simulink model "dpt"  (R2026a)
settings: Solver=ode23t  StopTime=simlength  FixedStep=tc  MaxStep=glb_time.tc  RelTol=1e-4
values from neighbouring files (symbols this model uses):
  afe_pwm_phase_shift_mod1 = 0    [init_model.m]
  glb_time = timing_setup(fpwm_afe, trgo_afe, fpwm_inv, trgo_inv, fpwm_single_phase_inv, trgo_single_phase_inv, fpwm_dab, trgo_dab,      fpwm_psfbc, trgo_psfbc, fpwm_isop_rail, trgo_isop_rail, fpwm_cllc, trgo_cllc, t_measure, tc_factor, tc_decimation, delay_pwm, dead_time_afe,      dead_time_inv, dead_time_single_phase_inv, dead_time_dab, dead_time_psfbc, dead_time_isop_rail, dead_time_cllc)    [init_model.m]
  time_gain_afe_module_1 = 1.0002    [init_model.m]
  time_gain_inv_module_2 = 1.001    [init_model.m]
libraries: fl_lib x18, nesl_utility x11, diode_rr_lib x2, igbt_dyn_lib x2, ee_lib x1, dclink_for_two_levels x1, single_phase_pwm_modulator x1
settings Model: Creator=dbagn  LastModifiedBy=dbagn
settings SolverCC: NumberNewtonIterations=3.0  ZeroCrossControl=DisableAll  SolverResetMethod=Robust
settings SFSimCC: CustomCodeUndefinedFunction=ThrowError  DefaultCustomCodeDeterministicFunctions=All
settings SFSimCC: SimCustomHeaderCode=|
  | #include "rpi.h"
  | #include "rpi_simulink.h"
  | #include "bemf_obsv_load_est.h"
  | #include "bemf_obsv_load_est_simulink.h"
  | #include "dqpll_grid.h"
  | #include "dsmavgflt.h"
  | #include "bemf_obsv.h"
  | #include "bemf_obsv_simulink.h"
  | #include "mavgflt.h"
  | #include "mavgflt_simulink.h"
  | #include "mavgflts.h"
  | #include "mavgflts_simulink.h"
  | #include "sv_pwm_cm.h"
  | #include "dsmavgflt_simulink.h"
  | #include "linear_double_integrator_observer_simulink.h"
  | #include "sv_pwm_cm_simulink.h"
  | #include "dqvector_pi.h"
  | #include "dqpll_grid_simulink.h"
  | #include "first_harmonic_tracker.h"
  | #include "dqvector_pi_simulink.h"
  | #include "first_harmonic_tracker_simulink.h"
  | #include "dqpll_thyr.h"
  | #include "sv_pwm_simulink.h"
  | #include "sv_pwm.h"
  | #include "dqpll_thyr_simulink.h"
  | #include "linear_double_integrator_observer.h"
  | #include "math_f.h"
settings SFSimCC: SimUserSources=|
  | "rpi.c"
  | "rpi_simulink.c"
  | "mavgflt_simulink.c"
  | "mavgflt.c"
  | "mavgflts_simulink.c"
  | "mavgflts.c"
  | "dsmavgflt_simulink.c"
  | "dsmavgflt.c"
  | "bemf_obsv_simulink.c"
  | "bemf_obsv.c"
  | "bemf_obsv_load_est_simulink.c"
  | "bemf_obsv_load_est.c"
  | "dqvector_pi.c"
  | "dqvector_pi_simulink.c"
  | "sv_pwm_simulink.c"
  | "sv_pwm.c"
  | "first_harmonic_tracker_simulink.c"
  | "first_harmonic_tracker.c"
  | "dqpll_thyr_simulink.c"
  | "dqpll_thyr.c"
  | "dqpll_grid_simulink.c"
  | "dqpll_grid.c"
  | "linear_double_integrator_observer_simulink.c"
  | "linear_double_integrator_observer.c"
  | "sv_pwm_cm_simulink.c"
  | "sv_pwm_cm.c"
settings SFSimCC: SimUserIncludeDirs=|
  | include
  | src
settings SimscapeCC: SimscapeNominalValues="[{\"value\":\"1\",\"unit\":\"A\"},{\"value\":\"1\",\"unit\":\"bar\"},{\"value\":\"1\",\"unit\":\"cm^2\"},{\"value\":\"1\",\"unit\":\"cm^3/s\"},{\"value\":\"1\",\"unit\":\"kJ/kg\"},{\"value\":\"1\",\"unit\":\"kW\"},{\"value\":\"1\",\"unit\":\"l\"},{\"value\":\"1\",\"unit\":\"N\"},{\"value\":\"1\",\"unit\":\"N*m\"},{\"value\":\"1\",\"unit\":\"V\"}]"  SimscapeLogType=none  SimscapeLogDataHistory=5000.0

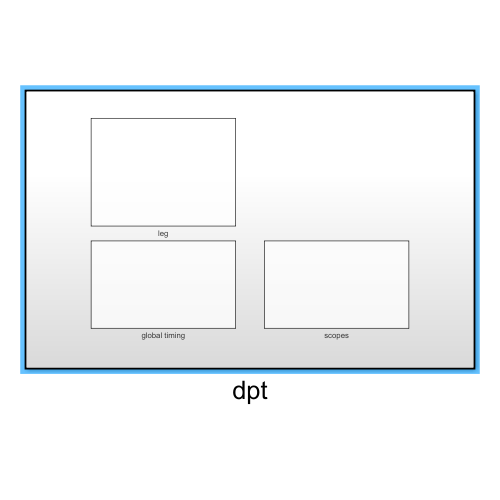
[thumbnail: Simulink's stored preview of the top-level diagram]
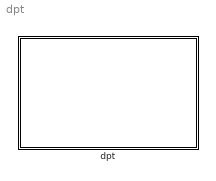
== system dpt ==
  dpt : Subsystem

== system dpt/dpt ==
  global timing : Subsystem
  leg : Subsystem
  scopes : Subsystem

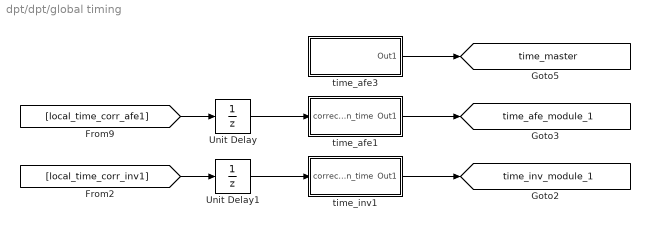
== system dpt/dpt/global timing ==
  Unit Delay : UnitDelay  SampleTime=glb_time.tc
  Unit Delay1 : UnitDelay  SampleTime=glb_time.tc
  time_afe1 : Subsystem  mask{k=time_gain_afe_module_1}
      mask prompts: k "Time Gain"
      mask Display:
      | disp('time-gen');
      | port_label('input', 1, 'crt');
      | port_label('output', 1, 'tout');
  time_afe3 : Subsystem  mask{k=1}
      mask prompts: k "Time Gain"
      mask Display:
      | disp('time-gen');
      | port_label('output', 1, 'tout');
  time_inv1 : Subsystem  mask{k=time_gain_inv_module_2}
      mask prompts: k "Time Gain"
      mask Display:
      | disp('time-gen');
      | port_label('input', 1, 'crt');
      | port_label('output', 1, 'tout');
  tag scope: time_afe_module_1=global, time_inv_module_1=global, time_master=global
  wires:
  Unit Delay1/1 -> time_inv1/1(correction_time)
  [local_time_corr_inv1] -> Unit Delay1/1
  Unit Delay/1 -> time_afe1/1(correction_time)
  [local_time_corr_afe1] -> Unit Delay/1
  time_afe3/1(Out1) -> [time_master]
  time_inv1/1(Out1) -> [time_inv_module_1]
  time_afe1/1(Out1) -> [time_afe_module_1]

== system dpt/dpt/leg ==
  Electrical Reference : fl_lib/Electrical/Electrical Elements/Electrical Reference
  Inductor : fl_lib/Electrical/Electrical Elements/Inductor  l=50e-6 H  r=0 Ohm  g=1e-9 1/Ohm  i_specify=off  i_priority=None  i=0 A  i_nominal_specify=off  i_nominal_value=1  i_nominal_unit=A  v_specify=off  v_priority=None  v=0 V  v_nominal_specify=off  v_nominal_value=1  v_nominal_unit=V  i_L_specify=off  i_L_priority=High  i_L=0 A  i_L_nominal_specify=off  i_L_nominal_value=1  i_L_nominal_unit=A
  Solver Configuration : nesl_utility/Solver Configuration  PhysicalDomain=network_engine_domain  SubClassName=solver  LeftPortType=input  RightPortType=generic  Tones=[]  Harmonics=[]  SimulateNoise=off  Profile=off  UseLocalSampling=off  EnableSwitchedLinearOptims=on  FrequencyDomain=off  UseCCode=off  RelTol=0.001  AbsTol=0.001  MinStep=1e-09  ToWorkspace=off  RevertToSquareIcSolve=off  NumHomotopyIterations=100  PhasorMode=off  PhasorModeNumHarmonics=1  ConsistencySolver=NEWTON_XTOL_AFTER_FTOL  CanonicalOrdering=CANONICAL  OptimizeIntermediates=OPTIMIZED  IndexReductionMethod=DerivativeReplacement  DoDC=off  ResidualTolerance=1e-09  ConsistencyTolSource=GLOBAL  ConsistencyAbsTol=0.001  ConsistencyRelTol=0.001  ConsistencyTolFactor=0.001  UseLocalSolver=off  LocalSolverChoice=NE_BACKWARD_EULER_ADVANCER  ResolveIndetEquations=on  FunctionEvalNumThread=1  LocalSolverSampleTime=glb_time.tc  DoFixedCost=off  MaxNonlinIter=nonlinear_iterations  MaxModeIter=2  ComputeImpulses=off  ImpulseIterations=2  LinearAlgebra=auto  LinearAlgebraNumThread=0  EquationFormulation=NE_TIME_EF  DelaysMemoryBudget=1024  AutomaticFiltering=on  FilteringTimeConstant=0.001  PartitionStorageMethod=AS_NEEDED  PartitionMemoryBudget=1024  PartitionMethod=ROBUST  MultibodyUseLocalSolver=off  MultibodyLocalSolverChoice=ODE1  MultibodyLocalSolverSampleTime=0.001
  Voltage Source : ee_lib/Sources/Voltage Source  dc_voltage=1070 V  ac_voltage=0 V  ac_shift=0 rad  ac_frequency=60 Hz  noise_mode=ee.enum.sources.noise.Disabled  PSD=0 V^2/Hz  sample_time=1e-3 s  repeatability=ee.enum.sources.repeatability.NotRepeatable  user_seed=0  auto_seed=2780181638  i_specify=off  i_priority=None  i=0 A  i_nominal_specify=off  i_nominal_value=1  i_nominal_unit=A  v_specify=off  v_priority=None  v=0 V  v_nominal_specify=off  v_nominal_value=1  v_nominal_unit=V
  leg : Subsystem
  connections:
  Voltage Source/RConn1 -- Solver Configuration/RConn1 -- Electrical Reference/LConn1 -- leg/RConn2
  Voltage Source/LConn1 -- leg/RConn1
  Inductor/LConn1 -- leg/LConn1
  Inductor/RConn1 -- leg/LConn2

== system dpt/dpt/scopes ==
  igbt_dyn : Subsystem

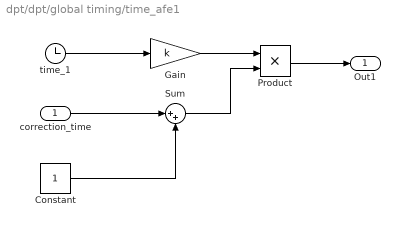
== system dpt/dpt/global timing/time_afe1 ==
  correction_time : Inport
  Constant : Constant
  Gain : Gain  Gain=k
  Product : Product
  Sum : Sum  Inputs=|++
  time_1 : Clock
  Out1 : Outport
  wires:
  Constant/1 -> Sum/2
  Sum/1 -> Product/2
  correction_time/1 -> Sum/1
  Product/1 -> Out1/1
  Gain/1 -> Product/1
  time_1/1 -> Gain/1

== system dpt/dpt/global timing/time_afe3 ==
  Gain : Gain  Gain=k
  time_1 : Clock
  Out1 : Outport
  wires:
  time_1/1 -> Gain/1
  Gain/1 -> Out1/1

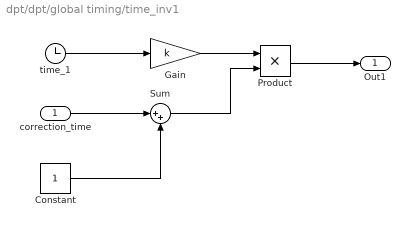
== system dpt/dpt/global timing/time_inv1 ==
  correction_time : Inport
  Constant : Constant
  Gain : Gain  Gain=k
  Product : Product
  Sum : Sum  Inputs=|++
  time_1 : Clock
  Out1 : Outport
  wires:
  Sum/1 -> Product/2
  Constant/1 -> Sum/2
  correction_time/1 -> Sum/1
  Product/1 -> Out1/1
  Gain/1 -> Product/1
  time_1/1 -> Gain/1

== system dpt/dpt/leg/leg ==
  dclink : Subsystem
  leg_pwm : Subsystem
  leg_with_igbt_dyn : Subsystem
  u1 : PMIOPort  Side=Left
  u2 : PMIOPort  Port=2  Side=Left
  Udc(+) : PMIOPort  Port=3  Side=Right
  Udc(-) : PMIOPort  Port=4  Side=Right
  wires:
  leg_pwm/1(gate_cmds) -> leg_with_igbt_dyn/1(gate_commands)
  connections:
  leg_with_igbt_dyn/RConn1 -- u1/RConn1
  leg_with_igbt_dyn/RConn2 -- u2/RConn1
  dclink/RConn1 -- Udc(+)/RConn1
  dclink/LConn1 -- leg_with_igbt_dyn/LConn1
  dclink/LConn2 -- leg_with_igbt_dyn/LConn2
  dclink/RConn2 -- Udc(-)/RConn1

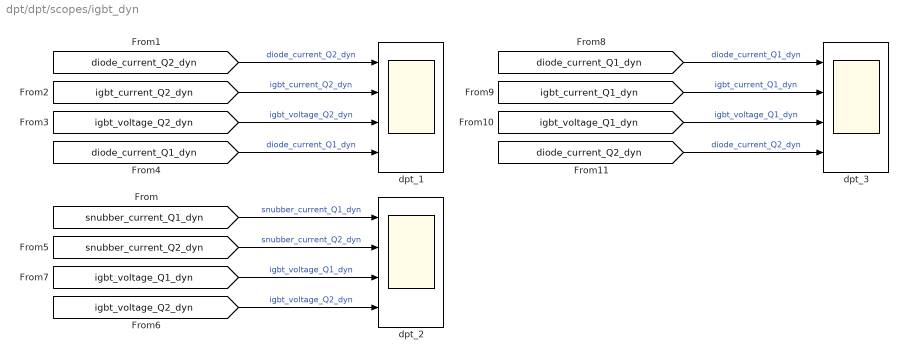
== system dpt/dpt/scopes/igbt_dyn ==
  dpt_1 : Scope  NumInputPorts=4
      settings: SampleTime=glb_time.tc  ActiveDisplayString=3  ActiveDisplayYMinimum=-199.00170924097591  ActiveDisplayYMaximum=1779.7216480499278
  dpt_2 : Scope  NumInputPorts=4
      settings: SampleTime=glb_time.tc  ActiveDisplayString=3  ActiveDisplayYMinimum=-153.38142747263524  ActiveDisplayYMaximum=1358.8196055613325
  dpt_3 : Scope  NumInputPorts=4
      settings: SampleTime=glb_time.tc  ActiveDisplayString=3  ActiveDisplayYMinimum=-153.38142747263524  ActiveDisplayYMaximum=1358.8196055613325  DataLoggingVariableName=ScopeData2
  wires:
  [diode_current_Q2_dyn] -> dpt_1/1  "diode_current_Q2_dyn"
  [igbt_voltage_Q2_dyn] -> dpt_1/3  "igbt_voltage_Q2_dyn"
  [igbt_current_Q2_dyn] -> dpt_1/2  "igbt_current_Q2_dyn"
  [diode_current_Q1_dyn] -> dpt_1/4  "diode_current_Q1_dyn"
  [snubber_current_Q1_dyn] -> dpt_2/1  "snubber_current_Q1_dyn"
  [snubber_current_Q2_dyn] -> dpt_2/2  "snubber_current_Q2_dyn"
  [igbt_voltage_Q2_dyn] -> dpt_2/4  "igbt_voltage_Q2_dyn"
  [igbt_voltage_Q1_dyn] -> dpt_2/3  "igbt_voltage_Q1_dyn"
  [diode_current_Q2_dyn] -> dpt_3/4  "diode_current_Q2_dyn"
  [igbt_current_Q1_dyn] -> dpt_3/2  "igbt_current_Q1_dyn"
  [igbt_voltage_Q1_dyn] -> dpt_3/3  "igbt_voltage_Q1_dyn"
  [diode_current_Q1_dyn] -> dpt_3/1  "diode_current_Q1_dyn"

== system dpt/dpt/leg/leg/dclink ==
  dclink1 : dclink_for_two_levels/dclink  Cdc=hwdata.afe.CFi  Rudc_measure=1e6  Vdc_scale=hwdata.afe.udc_nom
  Udc(+) : PMIOPort  Side=Right
  udc(+) : PMIOPort  Port=2  Side=Left
  udc(-) : PMIOPort  Port=3  Side=Left
  Udc(-) : PMIOPort  Port=4  Side=Right
  connections:
  dclink1/LConn2 -- udc(-)/RConn1
  dclink1/RConn2 -- Udc(-)/RConn1
  dclink1/RConn1 -- Udc(+)/RConn1
  dclink1/LConn1 -- udc(+)/RConn1

== system dpt/dpt/leg/leg/leg_pwm ==
  Constant1 : Constant  Value=afe_pwm_phase_shift_mod1
  Constant2 : Constant  Value=0.5
  modulator1 : Subsystem
  td2tc_1 : TransferFcn  Denominator=[glb_time.tc 1]
  gate_cmds : Outport
  wires:
  td2tc_1/1 -> modulator1/1(u)  "du(t)"
  Constant2/1 -> td2tc_1/1
  Constant1/1 -> modulator1/2(phase)
  modulator1/1(gate_cmds) -> gate_cmds/1

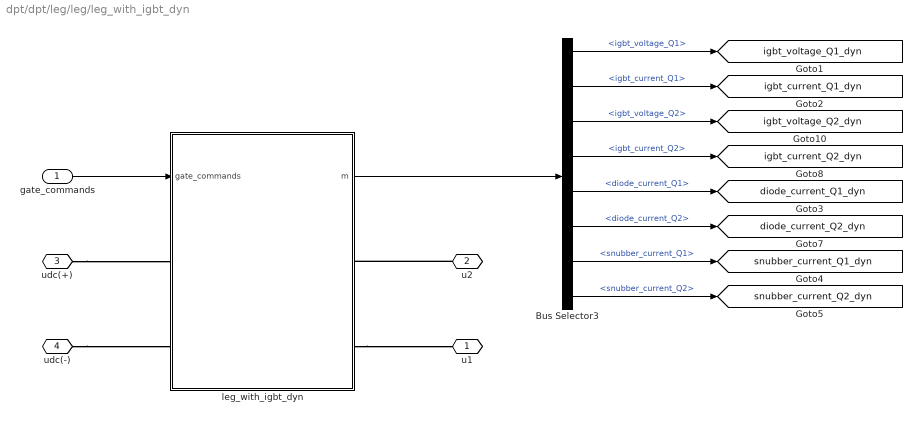
== system dpt/dpt/leg/leg/leg_with_igbt_dyn ==
  gate_commands : Inport
  Bus Selector3 : BusSelector  OutputSignals=igbt_voltage_Q1,igbt_current_Q1,igbt_voltage_Q2,igbt_current_Q2,diode_current_Q1,diode_current_Q2,snubber_current_Q1,snubber_current_Q2
  leg_with_igbt_dyn : Subsystem
  u1 : PMIOPort  Side=Right
  u2 : PMIOPort  Port=2  Side=Right
  udc(+) : PMIOPort  Port=3  Side=Left
  udc(-) : PMIOPort  Port=4  Side=Left
  tag scope: diode_current_Q1_dyn=global, diode_current_Q2_dyn=global, igbt_current_Q1_dyn=global, igbt_current_Q2_dyn=global, igbt_voltage_Q1_dyn=global, igbt_voltage_Q2_dyn=global, snubber_current_Q1_dyn=global, snubber_current_Q2_dyn=global
  wires:
  Bus Selector3/6 -> [diode_current_Q2_dyn]  "<diode_current_Q2>"
  Bus Selector3/5 -> [diode_current_Q1_dyn]  "<diode_current_Q1>"
  Bus Selector3/4 -> [igbt_current_Q2_dyn]  "<igbt_current_Q2>"
  Bus Selector3/3 -> [igbt_voltage_Q2_dyn]  "<igbt_voltage_Q2>"
  Bus Selector3/2 -> [igbt_current_Q1_dyn]  "<igbt_current_Q1>"
  Bus Selector3/1 -> [igbt_voltage_Q1_dyn]  "<igbt_voltage_Q1>"
  gate_commands/1 -> leg_with_igbt_dyn/1(gate_commands)
  leg_with_igbt_dyn/1(m) -> Bus Selector3/1
  Bus Selector3/7 -> [snubber_current_Q1_dyn]  "<snubber_current_Q1>"
  Bus Selector3/8 -> [snubber_current_Q2_dyn]  "<snubber_current_Q2>"
  connections:
  u2/RConn1 -- leg_with_igbt_dyn/RConn1
  udc(-)/RConn1 -- leg_with_igbt_dyn/LConn2
  udc(+)/RConn1 -- leg_with_igbt_dyn/LConn1
  leg_with_igbt_dyn/RConn2 -- u1/RConn1

== system dpt/dpt/leg/leg/leg_pwm/modulator1 ==
  u : Inport
  phase : Inport  Port=2
  one phase PWM generator with global TRGO : Subsystem  mask{f=glb_time.fPWM_AFE, m_up=0.98, m_low=0.02, dead_time=glb_time.dead_time_AFE, pos_cmd_gate=15, neg_cmd_gate=-8, polarity=1, tc=glb_time.tc, double_sampling=glb_time.TRGO_AFE_double_update}
      mask prompts: f "Frequency (Hz)"; m_up "Max Input Modulation Value"; m_low "Min Input Modulation Value"; dead_time "Dead Time (s)"; pos_cmd_gate "Positive Gate Voltage (V)"; neg_cmd_gate "Negative Gate Voltage (V)"; polarity "Polarity (pu)"; tc "Sampling time"
  gate_cmds : Outport
  wires:
  one phase PWM generator with global TRGO/2(gate_cmds) -> gate_cmds/1
  phase/1 -> one phase PWM generator with global TRGO/2(phase)
  u/1 -> one phase PWM generator with global TRGO/3(m)
  [time_afe_module_1] -> one phase PWM generator with global TRGO/1(time_source)

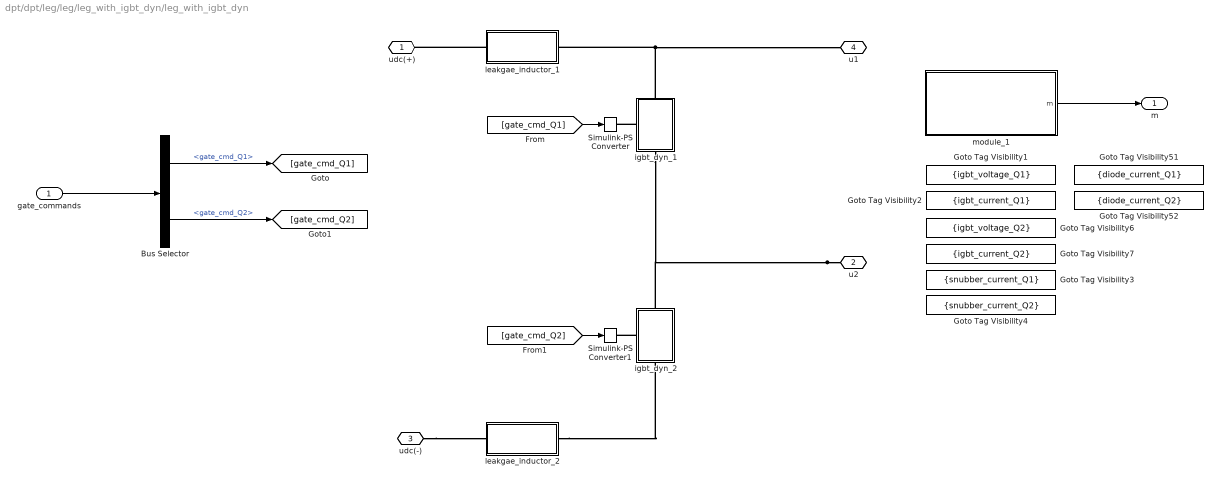
== system dpt/dpt/leg/leg/leg_with_igbt_dyn/leg_with_igbt_dyn ==
  gate_commands : Inport
  Bus Selector : BusSelector  OutputSignals=gate_cmd_Q1,gate_cmd_Q2
  Goto Tag Visibility1 : GotoTagVisibility  GotoTag=igbt_voltage_Q1
  Goto Tag Visibility2 : GotoTagVisibility  GotoTag=igbt_current_Q1
  Goto Tag Visibility3 : GotoTagVisibility  GotoTag=snubber_current_Q1
  Goto Tag Visibility4 : GotoTagVisibility  GotoTag=snubber_current_Q2
  Goto Tag Visibility51 : GotoTagVisibility  GotoTag=diode_current_Q1
  Goto Tag Visibility52 : GotoTagVisibility  GotoTag=diode_current_Q2
  Goto Tag Visibility6 : GotoTagVisibility  GotoTag=igbt_voltage_Q2
  Goto Tag Visibility7 : GotoTagVisibility  GotoTag=igbt_current_Q2
  Simulink-PS Converter : nesl_utility/Simulink-PS Converter  PhysicalDomain=network_engine_domain  SubClassName=ps_input  LeftPortType=input  RightPortType=output  PseudoPeriodic=off  Frequencies=[]  NoiseDistribution=none  NoiseParameters=[]  Unit=V  AffineConversion=off  FilteringAndDerivatives=provide  SimscapeFilterOrder=1  InputFilterTimeConstant=0.001  UdotUserProvided=0
  Simulink-PS Converter1 : nesl_utility/Simulink-PS Converter  PhysicalDomain=network_engine_domain  SubClassName=ps_input  LeftPortType=input  RightPortType=output  PseudoPeriodic=off  Frequencies=[]  NoiseDistribution=none  NoiseParameters=[]  Unit=V  AffineConversion=off  FilteringAndDerivatives=provide  SimscapeFilterOrder=1  InputFilterTimeConstant=0.001  UdotUserProvided=0
  igbt_dyn_1 : Subsystem
      settings: PortSchema="{\"entries\":[{\"content\":{\"sides\":[{\"content\":{\"connectorIds\":[\"LConn1\"]},\"type\":\"ConnectorPlacement.EquallySpacedRectSide\",\"uuid\":\"9277da8d-d460-43e6-8478-dd662f15d226\"},{\"content\":{\"connectorIds\":[],\"side\":\"RIGHT\"},\"type\":\"ConnectorPlacement.EquallySpacedRectSide\",\"uuid\":\"a7ece396-f1d9-4f4f-a05b-db1fc65d6e1d\"},{\"content\":{\"connectorIds\":[\"LConn2\"],\"side\":\"TOP\"},\"type\":\"ConnectorPlacement.EquallySpacedRectSide\",\"uuid\":\"fdd70777-e9cf-4317-afb6-cae87f75d5b0\"},{\"content\":{\"connectorIds\":[\"RConn1\"],\"side\":\"BOTTOM\"},\"type\":\"ConnectorPlacement.EquallySpacedRectSide\",\"uuid\":\"2353ed68-b1a1-4775-9ca9-31e268d5443b\"}]},\"type\":\"ConnectorPlacement.EquallySpacedConnector\",\"uuid\":\"d5479f4c-4e65-4791-adcb-73df11f88590\"}],\"packageUris\":[\"http://schema.mathworks.com/mf0/Connector/R2020b\"],\"version\":\"1.0\"}"
  igbt_dyn_2 : Subsystem
      settings: PortSchema="{\"entries\":[{\"content\":{\"sides\":[{\"content\":{\"connectorIds\":[\"LConn1\"]},\"type\":\"ConnectorPlacement.EquallySpacedRectSide\",\"uuid\":\"9277da8d-d460-43e6-8478-dd662f15d226\"},{\"content\":{\"connectorIds\":[],\"side\":\"RIGHT\"},\"type\":\"ConnectorPlacement.EquallySpacedRectSide\",\"uuid\":\"a7ece396-f1d9-4f4f-a05b-db1fc65d6e1d\"},{\"content\":{\"connectorIds\":[\"LConn2\"],\"side\":\"TOP\"},\"type\":\"ConnectorPlacement.EquallySpacedRectSide\",\"uuid\":\"fdd70777-e9cf-4317-afb6-cae87f75d5b0\"},{\"content\":{\"connectorIds\":[\"RConn1\"],\"side\":\"BOTTOM\"},\"type\":\"ConnectorPlacement.EquallySpacedRectSide\",\"uuid\":\"2353ed68-b1a1-4775-9ca9-31e268d5443b\"}]},\"type\":\"ConnectorPlacement.EquallySpacedConnector\",\"uuid\":\"d5479f4c-4e65-4791-adcb-73df11f88590\"}],\"packageUris\":[\"http://schema.mathworks.com/mf0/Connector/R2020b\"],\"version\":\"1.0\"}"
  leakgae_inductor_1 : Subsystem
  leakgae_inductor_2 : Subsystem
  module_1 : Subsystem
  udc(+) : PMIOPort  Side=Left
  u2 : PMIOPort  Port=2  Side=Right
  udc(-) : PMIOPort  Port=3  Side=Left
  u1 : PMIOPort  Port=4  Side=Right
  m : Outport
  wires:
  module_1/1(m) -> m/1
  Bus Selector/2 -> [gate_cmd_Q2]  "<gate_cmd_Q2>"
  Bus Selector/1 -> [gate_cmd_Q1]  "<gate_cmd_Q1>"
  [gate_cmd_Q2] -> Simulink-PS Converter1/1
  [gate_cmd_Q1] -> Simulink-PS Converter/1
  gate_commands/1 -> Bus Selector/1
  connections:
  igbt_dyn_2/LConn1 -- Simulink-PS Converter1/RConn1
  igbt_dyn_1/LConn1 -- Simulink-PS Converter/RConn1
  u2/RConn1 -- igbt_dyn_1/RConn1 -- igbt_dyn_2/LConn2
  leakgae_inductor_2/RConn1 -- igbt_dyn_2/RConn1
  igbt_dyn_1/LConn2 -- leakgae_inductor_1/RConn1 -- u1/RConn1
  udc(-)/RConn1 -- leakgae_inductor_2/LConn1
  leakgae_inductor_1/LConn1 -- udc(+)/RConn1

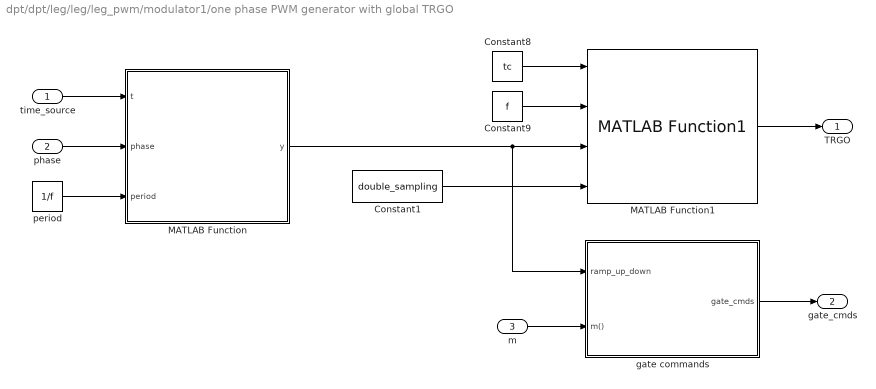
== system dpt/dpt/leg/leg/leg_pwm/modulator1/one phase PWM generator with global TRGO ==
  time_source : Inport
  phase : Inport  Port=2
  m : Inport  Port=3
  Constant1 : Constant  Value=double_sampling
  Constant8 : Constant  Value=tc
  Constant9 : Constant  Value=f
  MATLAB Function : MATLAB Function  TreatAsAtomicUnit=on  SystemSampleTime=tc
  MATLAB Function1 : single_phase_pwm_modulator/Single phase two level PWM generator with global TRGO/MATLAB Function1  SystemSampleTime=tc  VariantActivationTime=update diagram  EmptyChoice=off  PassThrough=off  PassThroughVariantControl=(default)  EmptyChoiceVariantControl=(default)  AllowFlexibleInterface=on  Latency=0  AutoFrameSizeCalculation=off
  gate commands : Subsystem
  period : Constant  Value=1/f
  TRGO : Outport
  gate_cmds : Outport  Port=2
  wires:
  period/1 -> MATLAB Function/3(period)
  phase/1 -> MATLAB Function/2(phase)
  MATLAB Function/1(y) -> gate commands/1(ramp_up_down), MATLAB Function1/3
  MATLAB Function1/1 -> TRGO/1
  Constant8/1 -> MATLAB Function1/1
  Constant9/1 -> MATLAB Function1/2
  m/1 -> gate commands/2(m())
  gate commands/1(gate_cmds) -> gate_cmds/1
  time_source/1 -> MATLAB Function/1(t)
  Constant1/1 -> MATLAB Function1/4

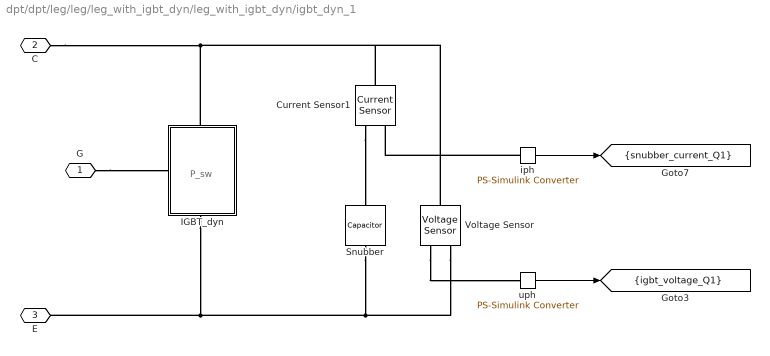
== system dpt/dpt/leg/leg/leg_with_igbt_dyn/leg_with_igbt_dyn/igbt_dyn_1 ==
  note: P_sw
  Current Sensor1 : fl_lib/Electrical/Electrical Sensors/Current Sensor
  IGBT_dyn : Subsystem
      settings: PortSchema="{\"entries\":[{\"content\":{\"sides\":[{\"content\":{\"connectorIds\":[\"LConn1\"]},\"type\":\"ConnectorPlacement.EquallySpacedRectSide\",\"uuid\":\"c3d88d60-081d-4221-ab18-079856838dba\"},{\"content\":{\"side\":\"RIGHT\"},\"type\":\"ConnectorPlacement.EquallySpacedRectSide\",\"uuid\":\"76e7d76c-8b60-4107-8aac-a7654bd886e1\"},{\"content\":{\"connectorIds\":[\"LConn2\"],\"side\":\"TOP\"},\"type\":\"ConnectorPlacement.EquallySpacedRectSide\",\"uuid\":\"fbef57e1-7143-4076-ada8-0654b1d9ee0b\"},{\"content\":{\"connectorIds\":[\"RConn1\"],\"side\":\"BOTTOM\"},\"type\":\"ConnectorPlacement.EquallySpacedRectSide\",\"uuid\":\"f2fea5db-9515-452a-a480-7d54bae36c49\"}]},\"type\":\"ConnectorPlacement.EquallySpacedConnector\",\"uuid\":\"cddff0b8-236e-4840-ad87-03abcdd65fe7\"}],\"packageUris\":[\"http://schema.mathworks.com/mf0/Connector/R2020b\"],\"version\":\"1.0\"}"
  Snubber : fl_lib/Electrical/Electrical Elements/Capacitor  c=igbt.afe.Csnubber_zvs F  r=igbt.afe.Rsnubber_zvs Ohm  g=0 1/Ohm  i_specify=off  i_priority=None  i=0 A  i_nominal_specify=off  i_nominal_value=1  i_nominal_unit=A  v_specify=off  v_priority=None  v=0 V  v_nominal_specify=off  v_nominal_value=1  v_nominal_unit=V  vc_specify=off  vc_priority=High  vc=0 V  vc_nominal_specify=off  vc_nominal_value=1  vc_nominal_unit=V
  Voltage Sensor : fl_lib/Electrical/Electrical Sensors/Voltage Sensor
  iph : nesl_utility/PS-Simulink Converter  PhysicalDomain=network_engine_domain  SubClassName=ps_output  LeftPortType=input  RightPortType=output  PseudoPeriodic=off  Frequencies=[]  VectorFormat=1-D array  Unit=A  AffineConversion=off
  uph : nesl_utility/PS-Simulink Converter  PhysicalDomain=network_engine_domain  SubClassName=ps_output  LeftPortType=input  RightPortType=output  PseudoPeriodic=off  Frequencies=[]  VectorFormat=1-D array  Unit=V  AffineConversion=off
  G : PMIOPort  Side=Left
  C : PMIOPort  Port=2  Side=Left
  E : PMIOPort  Port=3  Side=Right
  tag scope: igbt_voltage_Q1=scoped, snubber_current_Q1=scoped
  wires:
  uph/1 -> [igbt_voltage_Q1]
  iph/1 -> [snubber_current_Q1]
  connections:
  G/RConn1 -- IGBT_dyn/LConn1
  Voltage Sensor/RConn1 -- uph/LConn1
  IGBT_dyn/LConn2 -- Current Sensor1/LConn1 -- Voltage Sensor/LConn1 -- C/RConn1
  Voltage Sensor/RConn2 -- Snubber/RConn1 -- E/RConn1 -- IGBT_dyn/RConn1
  Current Sensor1/RConn2 -- Snubber/LConn1
  iph/LConn1 -- Current Sensor1/RConn1

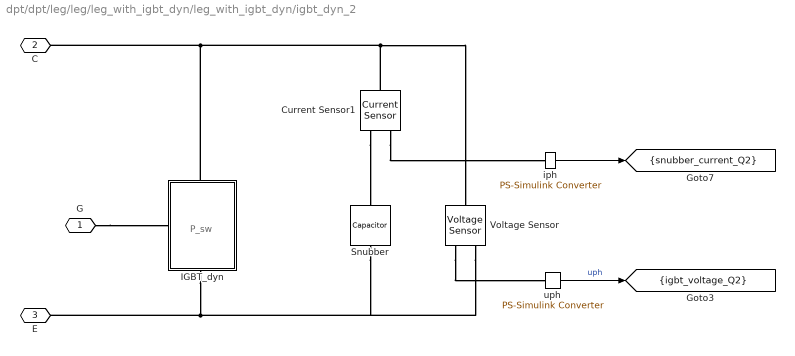
== system dpt/dpt/leg/leg/leg_with_igbt_dyn/leg_with_igbt_dyn/igbt_dyn_2 ==
  note: P_sw
  Current Sensor1 : fl_lib/Electrical/Electrical Sensors/Current Sensor
  IGBT_dyn : Subsystem
      settings: PortSchema="{\"entries\":[{\"content\":{\"sides\":[{\"content\":{\"connectorIds\":[\"LConn1\"]},\"type\":\"ConnectorPlacement.EquallySpacedRectSide\",\"uuid\":\"c3d88d60-081d-4221-ab18-079856838dba\"},{\"content\":{\"side\":\"RIGHT\"},\"type\":\"ConnectorPlacement.EquallySpacedRectSide\",\"uuid\":\"76e7d76c-8b60-4107-8aac-a7654bd886e1\"},{\"content\":{\"connectorIds\":[\"LConn2\"],\"side\":\"TOP\"},\"type\":\"ConnectorPlacement.EquallySpacedRectSide\",\"uuid\":\"fbef57e1-7143-4076-ada8-0654b1d9ee0b\"},{\"content\":{\"connectorIds\":[\"RConn1\"],\"side\":\"BOTTOM\"},\"type\":\"ConnectorPlacement.EquallySpacedRectSide\",\"uuid\":\"f2fea5db-9515-452a-a480-7d54bae36c49\"}]},\"type\":\"ConnectorPlacement.EquallySpacedConnector\",\"uuid\":\"cddff0b8-236e-4840-ad87-03abcdd65fe7\"}],\"packageUris\":[\"http://schema.mathworks.com/mf0/Connector/R2020b\"],\"version\":\"1.0\"}"
  Snubber : fl_lib/Electrical/Electrical Elements/Capacitor  c=igbt.afe.Csnubber_zvs F  r=igbt.afe.Rsnubber_zvs Ohm  g=0 1/Ohm  i_specify=off  i_priority=None  i=0 A  i_nominal_specify=off  i_nominal_value=1  i_nominal_unit=A  v_specify=off  v_priority=None  v=0 V  v_nominal_specify=off  v_nominal_value=1  v_nominal_unit=V  vc_specify=off  vc_priority=High  vc=0 V  vc_nominal_specify=off  vc_nominal_value=1  vc_nominal_unit=V
  Voltage Sensor : fl_lib/Electrical/Electrical Sensors/Voltage Sensor
  iph : nesl_utility/PS-Simulink Converter  PhysicalDomain=network_engine_domain  SubClassName=ps_output  LeftPortType=input  RightPortType=output  PseudoPeriodic=off  Frequencies=[]  VectorFormat=1-D array  Unit=A  AffineConversion=off
  uph : nesl_utility/PS-Simulink Converter  PhysicalDomain=network_engine_domain  SubClassName=ps_output  LeftPortType=input  RightPortType=output  PseudoPeriodic=off  Frequencies=[]  VectorFormat=1-D array  Unit=V  AffineConversion=off
  G : PMIOPort  Side=Left
  C : PMIOPort  Port=2  Side=Left
  E : PMIOPort  Port=3  Side=Right
  tag scope: igbt_voltage_Q2=scoped, snubber_current_Q2=scoped
  wires:
  uph/1 -> [igbt_voltage_Q2]  "uph"
  iph/1 -> [snubber_current_Q2]
  connections:
  IGBT_dyn/RConn1 -- Voltage Sensor/RConn2 -- Snubber/RConn1 -- E/RConn1
  Voltage Sensor/RConn1 -- uph/LConn1
  G/RConn1 -- IGBT_dyn/LConn1
  Current Sensor1/RConn2 -- Snubber/LConn1
  Current Sensor1/RConn1 -- iph/LConn1
  Current Sensor1/LConn1 -- Voltage Sensor/LConn1 -- IGBT_dyn/LConn2 -- C/RConn1

== system dpt/dpt/leg/leg/leg_with_igbt_dyn/leg_with_igbt_dyn/leakgae_inductor_1 ==
  Inductor : fl_lib/Electrical/Electrical Elements/Inductor  l=10e-9 H  r=5e-3 Ohm  g=1e-9 1/Ohm  i_specify=off  i_priority=None  i=0 A  i_nominal_specify=off  i_nominal_value=1  i_nominal_unit=A  v_specify=off  v_priority=None  v=0 V  v_nominal_specify=off  v_nominal_value=1  v_nominal_unit=V  i_L_specify=off  i_L_priority=High  i_L=0 A  i_L_nominal_specify=off  i_L_nominal_value=1  i_L_nominal_unit=A
  Resistor : fl_lib/Electrical/Electrical Elements/Resistor  R=1 Ohm  i_specify=off  i_priority=None  i=0 A  i_nominal_specify=off  i_nominal_value=1  i_nominal_unit=A  v_specify=off  v_priority=None  v=0 V  v_nominal_specify=off  v_nominal_value=1  v_nominal_unit=V
  in : PMIOPort  Side=Left
  out : PMIOPort  Port=2  Side=Right
  connections:
  Resistor/RConn1 -- Inductor/RConn1 -- out/RConn1
  Resistor/LConn1 -- Inductor/LConn1 -- in/RConn1

== system dpt/dpt/leg/leg/leg_with_igbt_dyn/leg_with_igbt_dyn/leakgae_inductor_2 ==
  Inductor : fl_lib/Electrical/Electrical Elements/Inductor  l=10e-9 H  r=5e-3 Ohm  g=1e-9 1/Ohm  i_specify=off  i_priority=None  i=0 A  i_nominal_specify=off  i_nominal_value=1  i_nominal_unit=A  v_specify=off  v_priority=None  v=0 V  v_nominal_specify=off  v_nominal_value=1  v_nominal_unit=V  i_L_specify=off  i_L_priority=High  i_L=0 A  i_L_nominal_specify=off  i_L_nominal_value=1  i_L_nominal_unit=A
  Resistor : fl_lib/Electrical/Electrical Elements/Resistor  R=1 Ohm  i_specify=off  i_priority=None  i=0 A  i_nominal_specify=off  i_nominal_value=1  i_nominal_unit=A  v_specify=off  v_priority=None  v=0 V  v_nominal_specify=off  v_nominal_value=1  v_nominal_unit=V
  in : PMIOPort  Side=Left
  out : PMIOPort  Port=2  Side=Right
  connections:
  in/RConn1 -- Inductor/LConn1 -- Resistor/LConn1
  out/RConn1 -- Inductor/RConn1 -- Resistor/RConn1

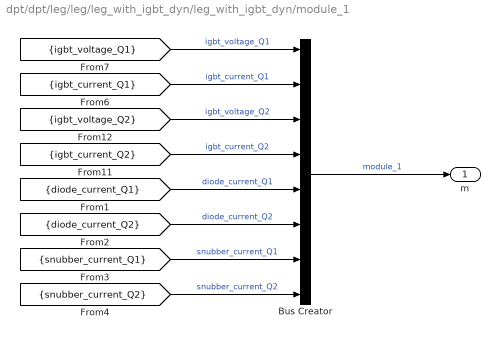
== system dpt/dpt/leg/leg/leg_with_igbt_dyn/leg_with_igbt_dyn/module_1 ==
  Bus Creator : BusCreator  Inputs=8
  m : Outport
  wires:
  [igbt_current_Q1] -> Bus Creator/2  "igbt_current_Q1"
  [igbt_voltage_Q1] -> Bus Creator/1  "igbt_voltage_Q1"
  [igbt_voltage_Q2] -> Bus Creator/3  "igbt_voltage_Q2"
  [igbt_current_Q2] -> Bus Creator/4  "igbt_current_Q2"
  Bus Creator/1 -> m/1  "module_1"
  [diode_current_Q1] -> Bus Creator/5  "diode_current_Q1"
  [diode_current_Q2] -> Bus Creator/6  "diode_current_Q2"
  [snubber_current_Q1] -> Bus Creator/7  "snubber_current_Q1"
  [snubber_current_Q2] -> Bus Creator/8  "snubber_current_Q2"

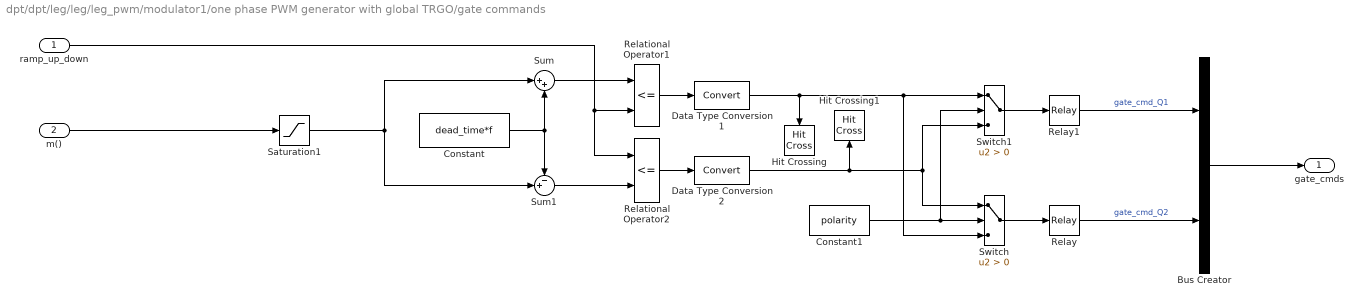
== system dpt/dpt/leg/leg/leg_pwm/modulator1/one phase PWM generator with global TRGO/gate commands ==
  ramp_up_down : Inport
  m() : Inport  Port=2
  Bus Creator : BusCreator  Inputs=2
  Constant : Constant  Value=dead_time*f
  Constant1 : Constant  Value=polarity
  Data Type Conversion1 : DataTypeConversion
  Data Type Conversion2 : DataTypeConversion
  Hit Crossing : HitCross  ShowOutputPort=off
  Hit Crossing1 : HitCross  ShowOutputPort=off
  Relational Operator1 : RelationalOperator  Operator=<=  InputSameDT=off
  Relational Operator2 : RelationalOperator  Operator=<=  InputSameDT=off
  Relay : Relay  OnOutputValue=pos_cmd_gate  OffOutputValue=neg_cmd_gate
  Relay1 : Relay  OnOutputValue=pos_cmd_gate  OffOutputValue=neg_cmd_gate
  Saturation1 : Saturate  UpperLimit=m_up  LowerLimit=m_low
  Sum : Sum  Inputs=|++  SaturateOnIntegerOverflow=on
  Sum1 : Sum  Inputs=-+|  SaturateOnIntegerOverflow=on
  Switch : Switch  Criteria=u2 > Threshold  SaturateOnIntegerOverflow=off  InputSameDT=off
  Switch1 : Switch  Criteria=u2 > Threshold  SaturateOnIntegerOverflow=off  InputSameDT=off
  gate_cmds : Outport
  wires:
  Constant1/1 -> Switch1/2, Switch/2
  Data Type Conversion1/1 -> Switch/3, Switch1/1, Hit Crossing/1
  Saturation1/1 -> Sum1/2, Sum/1
  Data Type Conversion2/1 -> Switch/1, Switch1/3, Hit Crossing1/1
  Relational Operator1/1 -> Data Type Conversion1/1
  Bus Creator/1 -> gate_cmds/1
  Sum1/1 -> Relational Operator2/2
  Switch/1 -> Relay/1
  Sum/1 -> Relational Operator1/1
  m()/1 -> Saturation1/1
  ramp_up_down/1 -> Relational Operator2/1, Relational Operator1/2
  Switch1/1 -> Relay1/1
  Relational Operator2/1 -> Data Type Conversion2/1
  Relay/1 -> Bus Creator/2  "gate_cmd_Q2"
  Relay1/1 -> Bus Creator/1  "gate_cmd_Q1"
  Constant/1 -> Sum/2, Sum1/1

== system dpt/dpt/leg/leg/leg_with_igbt_dyn/leg_with_igbt_dyn/igbt_dyn_1/IGBT_dyn ==
  Diode_rr : Subsystem
      settings: PortSchema="{\"entries\":[{\"content\":{\"sides\":[{\"content\":{},\"type\":\"ConnectorPlacement.EquallySpacedRectSide\",\"uuid\":\"771776bd-f835-4cc9-abb3-440f51d02f91\"},{\"content\":{\"side\":\"RIGHT\"},\"type\":\"ConnectorPlacement.EquallySpacedRectSide\",\"uuid\":\"78ab2f96-400e-4671-b13c-5de3303ef4f0\"},{\"content\":{\"connectorIds\":[\"LConn1\"],\"side\":\"TOP\"},\"type\":\"ConnectorPlacement.EquallySpacedRectSide\",\"uuid\":\"8ca13711-c5a2-4f63-b70d-8d380fc192f5\"},{\"content\":{\"connectorIds\":[\"RConn1\"],\"side\":\"BOTTOM\"},\"type\":\"ConnectorPlacement.EquallySpacedRectSide\",\"uuid\":\"2a5f65ce-9e27-46ac-9ba5-1ee8508da976\"}]},\"type\":\"ConnectorPlacement.EquallySpacedConnector\",\"uuid\":\"3750f3f3-140e-42a5-b17d-41831cba29de\"}],\"packageUris\":[\"http://schema.mathworks.com/mf0/Connector/R2020b\"],\"version\":\"1.0\"}"
  IGBT_dyn : Subsystem
      settings: PortSchema="{\"entries\":[{\"content\":{\"sides\":[{\"content\":{},\"type\":\"ConnectorPlacement.EquallySpacedRectSide\",\"uuid\":\"84b34275-d607-4bea-822f-0dba7f36167f\"},{\"content\":{\"connectorIds\":[\"RConn1\"],\"side\":\"RIGHT\"},\"type\":\"ConnectorPlacement.EquallySpacedRectSide\",\"uuid\":\"6edccc11-9562-49ee-afd6-b8e577eb322e\"},{\"content\":{\"connectorIds\":[\"LConn1\"],\"side\":\"TOP\"},\"type\":\"ConnectorPlacement.EquallySpacedRectSide\",\"uuid\":\"046a6cea-8aaa-4489-a02e-7ffcc409a169\"},{\"content\":{\"connectorIds\":[\"RConn2\"],\"side\":\"BOTTOM\"},\"type\":\"ConnectorPlacement.EquallySpacedRectSide\",\"uuid\":\"e0630a31-429d-401d-96bb-6f7299452ccc\"}]},\"type\":\"ConnectorPlacement.EquallySpacedConnector\",\"uuid\":\"d17d1ed5-06f3-484d-96a8-b04d1c367457\"}],\"packageUris\":[\"http://schema.mathworks.com/mf0/Connector/R2020b\"],\"version\":\"1.0\"}"
  G : PMIOPort  Side=Left
  C : PMIOPort  Port=2  Side=Left
  E : PMIOPort  Port=3  Side=Right
  connections:
  C/RConn1 -- Diode_rr/LConn1 -- IGBT_dyn/LConn1
  IGBT_dyn/RConn2 -- Diode_rr/RConn1 -- E/RConn1
  IGBT_dyn/RConn1 -- G/RConn1

== system dpt/dpt/leg/leg/leg_with_igbt_dyn/leg_with_igbt_dyn/igbt_dyn_2/IGBT_dyn ==
  Diode_rr : Subsystem
      settings: PortSchema="{\"entries\":[{\"content\":{\"sides\":[{\"content\":{},\"type\":\"ConnectorPlacement.EquallySpacedRectSide\",\"uuid\":\"771776bd-f835-4cc9-abb3-440f51d02f91\"},{\"content\":{\"side\":\"RIGHT\"},\"type\":\"ConnectorPlacement.EquallySpacedRectSide\",\"uuid\":\"78ab2f96-400e-4671-b13c-5de3303ef4f0\"},{\"content\":{\"connectorIds\":[\"LConn1\"],\"side\":\"TOP\"},\"type\":\"ConnectorPlacement.EquallySpacedRectSide\",\"uuid\":\"8ca13711-c5a2-4f63-b70d-8d380fc192f5\"},{\"content\":{\"connectorIds\":[\"RConn1\"],\"side\":\"BOTTOM\"},\"type\":\"ConnectorPlacement.EquallySpacedRectSide\",\"uuid\":\"2a5f65ce-9e27-46ac-9ba5-1ee8508da976\"}]},\"type\":\"ConnectorPlacement.EquallySpacedConnector\",\"uuid\":\"3750f3f3-140e-42a5-b17d-41831cba29de\"}],\"packageUris\":[\"http://schema.mathworks.com/mf0/Connector/R2020b\"],\"version\":\"1.0\"}"
  IGBT_dyn : Subsystem
      settings: PortSchema="{\"entries\":[{\"content\":{\"sides\":[{\"content\":{},\"type\":\"ConnectorPlacement.EquallySpacedRectSide\",\"uuid\":\"84b34275-d607-4bea-822f-0dba7f36167f\"},{\"content\":{\"connectorIds\":[\"RConn1\"],\"side\":\"RIGHT\"},\"type\":\"ConnectorPlacement.EquallySpacedRectSide\",\"uuid\":\"6edccc11-9562-49ee-afd6-b8e577eb322e\"},{\"content\":{\"connectorIds\":[\"LConn1\"],\"side\":\"TOP\"},\"type\":\"ConnectorPlacement.EquallySpacedRectSide\",\"uuid\":\"046a6cea-8aaa-4489-a02e-7ffcc409a169\"},{\"content\":{\"connectorIds\":[\"RConn2\"],\"side\":\"BOTTOM\"},\"type\":\"ConnectorPlacement.EquallySpacedRectSide\",\"uuid\":\"e0630a31-429d-401d-96bb-6f7299452ccc\"}]},\"type\":\"ConnectorPlacement.EquallySpacedConnector\",\"uuid\":\"d17d1ed5-06f3-484d-96a8-b04d1c367457\"}],\"packageUris\":[\"http://schema.mathworks.com/mf0/Connector/R2020b\"],\"version\":\"1.0\"}"
  G : PMIOPort  Side=Left
  C : PMIOPort  Port=2  Side=Left
  E : PMIOPort  Port=3  Side=Right
  connections:
  IGBT_dyn/RConn1 -- G/RConn1
  Diode_rr/RConn1 -- E/RConn1 -- IGBT_dyn/RConn2
  Diode_rr/LConn1 -- IGBT_dyn/LConn1 -- C/RConn1

== system dpt/dpt/leg/leg/leg_with_igbt_dyn/leg_with_igbt_dyn/igbt_dyn_1/IGBT_dyn/Diode_rr ==
  Current Sensor1 : fl_lib/Electrical/Electrical Sensors/Current Sensor
  diode_rr : Subsystem
  iph2 : nesl_utility/PS-Simulink Converter  PhysicalDomain=network_engine_domain  SubClassName=ps_output  LeftPortType=input  RightPortType=output  PseudoPeriodic=off  Frequencies=[]  VectorFormat=1-D array  Unit=A  AffineConversion=off
  K : PMIOPort  Side=Left
  A : PMIOPort  Port=2  Side=Right
  tag scope: diode_current_Q1=scoped
  wires:
  iph2/1 -> [diode_current_Q1]  "i_device_thermal_inv"
  connections:
  diode_rr/LConn1 -- A/RConn1
  diode_rr/RConn1 -- Current Sensor1/RConn2
  iph2/LConn1 -- Current Sensor1/RConn1
  K/RConn1 -- Current Sensor1/LConn1

== system dpt/dpt/leg/leg/leg_with_igbt_dyn/leg_with_igbt_dyn/igbt_dyn_1/IGBT_dyn/IGBT_dyn ==
  Controlled Voltage Source : fl_lib/Electrical/Electrical Sources/Controlled Voltage Source
  IGBT_dyn : Subsystem
      settings: PortSchema="{\"entries\":[{\"content\":{\"sides\":[{\"content\":{\"connectorIds\":[\"LConn1\"]},\"type\":\"ConnectorPlacement.EquallySpacedRectSide\",\"uuid\":\"84b34275-d607-4bea-822f-0dba7f36167f\"},{\"content\":{\"side\":\"RIGHT\"},\"type\":\"ConnectorPlacement.EquallySpacedRectSide\",\"uuid\":\"6edccc11-9562-49ee-afd6-b8e577eb322e\"},{\"content\":{\"connectorIds\":[\"LConn2\"],\"side\":\"TOP\"},\"type\":\"ConnectorPlacement.EquallySpacedRectSide\",\"uuid\":\"046a6cea-8aaa-4489-a02e-7ffcc409a169\"},{\"content\":{\"connectorIds\":[\"RConn1\"],\"side\":\"BOTTOM\"},\"type\":\"ConnectorPlacement.EquallySpacedRectSide\",\"uuid\":\"59c08e69-e271-4d9d-819b-a93d614eacb6\"}]},\"type\":\"ConnectorPlacement.EquallySpacedConnector\",\"uuid\":\"d17d1ed5-06f3-484d-96a8-b04d1c367457\"}],\"packageUris\":[\"http://schema.mathworks.com/mf0/Connector/R2020b\"],\"version\":\"1.0\"}"
  C : PMIOPort  Side=Left
  G : PMIOPort  Port=2  Side=Right
  E : PMIOPort  Port=3  Side=Right
  connections:
  Controlled Voltage Source/LConn1 -- IGBT_dyn/LConn1
  Controlled Voltage Source/RConn1 -- G/RConn1
  E/RConn1 -- IGBT_dyn/RConn1 -- Controlled Voltage Source/RConn2
  C/RConn1 -- IGBT_dyn/LConn2

== system dpt/dpt/leg/leg/leg_with_igbt_dyn/leg_with_igbt_dyn/igbt_dyn_2/IGBT_dyn/Diode_rr ==
  Current Sensor1 : fl_lib/Electrical/Electrical Sensors/Current Sensor
  diode_rr : Subsystem
  iph2 : nesl_utility/PS-Simulink Converter  PhysicalDomain=network_engine_domain  SubClassName=ps_output  LeftPortType=input  RightPortType=output  PseudoPeriodic=off  Frequencies=[]  VectorFormat=1-D array  Unit=A  AffineConversion=off
  K : PMIOPort  Side=Left
  A : PMIOPort  Port=2  Side=Right
  tag scope: diode_current_Q2=scoped
  wires:
  iph2/1 -> [diode_current_Q2]  "i_device_thermal_inv"
  connections:
  K/RConn1 -- Current Sensor1/LConn1
  iph2/LConn1 -- Current Sensor1/RConn1
  diode_rr/RConn1 -- Current Sensor1/RConn2
  diode_rr/LConn1 -- A/RConn1

== system dpt/dpt/leg/leg/leg_with_igbt_dyn/leg_with_igbt_dyn/igbt_dyn_2/IGBT_dyn/IGBT_dyn ==
  Controlled Voltage Source : fl_lib/Electrical/Electrical Sources/Controlled Voltage Source
  IGBT_dyn : Subsystem
      settings: PortSchema="{\"entries\":[{\"content\":{\"sides\":[{\"content\":{\"connectorIds\":[\"LConn1\"]},\"type\":\"ConnectorPlacement.EquallySpacedRectSide\",\"uuid\":\"84b34275-d607-4bea-822f-0dba7f36167f\"},{\"content\":{\"side\":\"RIGHT\"},\"type\":\"ConnectorPlacement.EquallySpacedRectSide\",\"uuid\":\"6edccc11-9562-49ee-afd6-b8e577eb322e\"},{\"content\":{\"connectorIds\":[\"LConn2\"],\"side\":\"TOP\"},\"type\":\"ConnectorPlacement.EquallySpacedRectSide\",\"uuid\":\"046a6cea-8aaa-4489-a02e-7ffcc409a169\"},{\"content\":{\"connectorIds\":[\"RConn1\"],\"side\":\"BOTTOM\"},\"type\":\"ConnectorPlacement.EquallySpacedRectSide\",\"uuid\":\"59c08e69-e271-4d9d-819b-a93d614eacb6\"}]},\"type\":\"ConnectorPlacement.EquallySpacedConnector\",\"uuid\":\"d17d1ed5-06f3-484d-96a8-b04d1c367457\"}],\"packageUris\":[\"http://schema.mathworks.com/mf0/Connector/R2020b\"],\"version\":\"1.0\"}"
  C : PMIOPort  Side=Left
  G : PMIOPort  Port=2  Side=Right
  E : PMIOPort  Port=3  Side=Right
  connections:
  C/RConn1 -- IGBT_dyn/LConn2
  IGBT_dyn/RConn1 -- E/RConn1 -- Controlled Voltage Source/RConn2
  Controlled Voltage Source/RConn1 -- G/RConn1
  Controlled Voltage Source/LConn1 -- IGBT_dyn/LConn1

== system dpt/dpt/leg/leg/leg_with_igbt_dyn/leg_with_igbt_dyn/igbt_dyn_1/IGBT_dyn/Diode_rr/diode_rr ==
  RR Diode (Lauritzen-Ma) : diode_rr_lib/RR Diode (Lauritzen-Ma)  Is=5e-9 A  N=2  Vt=26e-3 V  tau=350e-9 s  TM=60e-9 s  Rs=0.5e-3 Ohm  Cj0=10e-9 F  Vjp=0.7 V  mg=0.5  FC=0.5  dsm=0.1 V  i_specify=off  i_priority=None  i=0 A  i_nominal_specify=off  i_nominal_value=1  i_nominal_unit=A  v_specify=off  v_priority=None  v=0 V  v_nominal_specify=off  v_nominal_value=1  v_nominal_unit=V  vj_specify=off  vj_priority=None  vj=0 V  vj_nominal_specify=off  vj_nominal_value=1  vj_nominal_unit=V  qE_specify=off  qE_priority=None  qE=0 C  qE_nominal_specify=off  qE_nominal_value=1  qE_nominal_unit=C  qM_specify=off  qM_priority=High  qM=0 C  qM_nominal_specify=off  qM_nominal_value=1  qM_nominal_unit=C  qj_specify=off  qj_priority=None  qj=0 C  qj_nominal_specify=off  qj_nominal_value=1  qj_nominal_unit=C
  A : PMIOPort  Side=Left
  K : PMIOPort  Port=2  Side=Right
  connections:
  RR Diode (Lauritzen-Ma)/LConn1 -- A/RConn1
  RR Diode (Lauritzen-Ma)/RConn1 -- K/RConn1

== system dpt/dpt/leg/leg/leg_with_igbt_dyn/leg_with_igbt_dyn/igbt_dyn_1/IGBT_dyn/IGBT_dyn/IGBT_dyn ==
  Current Sensor : fl_lib/Electrical/Electrical Sensors/Current Sensor
  igbt_dyn : Subsystem
      settings: PortSchema="{\"entries\":[{\"content\":{\"sides\":[{\"content\":{\"connectorIds\":[\"LConn1\"]},\"type\":\"ConnectorPlacement.EquallySpacedRectSide\",\"uuid\":\"9362f9b7-ee93-45f5-82dd-187a901e7163\"},{\"content\":{\"side\":\"RIGHT\"},\"type\":\"ConnectorPlacement.EquallySpacedRectSide\",\"uuid\":\"6bcfd024-782a-41e2-b73d-7f1803740400\"},{\"content\":{\"connectorIds\":[\"LConn2\"],\"side\":\"TOP\"},\"type\":\"ConnectorPlacement.EquallySpacedRectSide\",\"uuid\":\"acf2fd2a-16ab-451c-9949-ad592b9336db\"},{\"content\":{\"connectorIds\":[\"RConn1\"],\"side\":\"BOTTOM\"},\"type\":\"ConnectorPlacement.EquallySpacedRectSide\",\"uuid\":\"befa74e7-1b93-47d7-b2f5-8e4e16cc48d3\"}]},\"type\":\"ConnectorPlacement.EquallySpacedConnector\",\"uuid\":\"1ef05993-5e93-4d63-8a9c-9607affd4d31\"}],\"packageUris\":[\"http://schema.mathworks.com/mf0/Connector/R2020b\"],\"version\":\"1.0\"}"
  iph1 : nesl_utility/PS-Simulink Converter  PhysicalDomain=network_engine_domain  SubClassName=ps_output  LeftPortType=input  RightPortType=output  PseudoPeriodic=off  Frequencies=[]  VectorFormat=1-D array  Unit=A  AffineConversion=off
  G : PMIOPort  Side=Left
  C : PMIOPort  Port=2  Side=Left
  E : PMIOPort  Port=3  Side=Right
  tag scope: igbt_current_Q1=scoped
  wires:
  iph1/1 -> [igbt_current_Q1]  "i_device_thermal_inv"
  connections:
  G/RConn1 -- igbt_dyn/LConn1
  iph1/LConn1 -- Current Sensor/RConn1
  Current Sensor/RConn2 -- igbt_dyn/LConn2
  E/RConn1 -- igbt_dyn/RConn1
  C/RConn1 -- Current Sensor/LConn1

== system dpt/dpt/leg/leg/leg_with_igbt_dyn/leg_with_igbt_dyn/igbt_dyn_2/IGBT_dyn/Diode_rr/diode_rr ==
  RR Diode (Lauritzen-Ma) : diode_rr_lib/RR Diode (Lauritzen-Ma)  Is=5e-9 A  N=2  Vt=26e-3 V  tau=350e-9 s  TM=60e-9 s  Rs=0.5e-3 Ohm  Cj0=10e-9 F  Vjp=0.7 V  mg=0.5  FC=0.5  dsm=0.1 V  i_specify=off  i_priority=None  i=0 A  i_nominal_specify=off  i_nominal_value=1  i_nominal_unit=A  v_specify=off  v_priority=None  v=0 V  v_nominal_specify=off  v_nominal_value=1  v_nominal_unit=V  vj_specify=off  vj_priority=None  vj=0 V  vj_nominal_specify=off  vj_nominal_value=1  vj_nominal_unit=V  qE_specify=off  qE_priority=None  qE=0 C  qE_nominal_specify=off  qE_nominal_value=1  qE_nominal_unit=C  qM_specify=off  qM_priority=High  qM=0 C  qM_nominal_specify=off  qM_nominal_value=1  qM_nominal_unit=C  qj_specify=off  qj_priority=None  qj=0 C  qj_nominal_specify=off  qj_nominal_value=1  qj_nominal_unit=C
  A : PMIOPort  Side=Left
  K : PMIOPort  Port=2  Side=Right
  connections:
  RR Diode (Lauritzen-Ma)/RConn1 -- K/RConn1
  RR Diode (Lauritzen-Ma)/LConn1 -- A/RConn1

== system dpt/dpt/leg/leg/leg_with_igbt_dyn/leg_with_igbt_dyn/igbt_dyn_2/IGBT_dyn/IGBT_dyn/IGBT_dyn ==
  Current Sensor : fl_lib/Electrical/Electrical Sensors/Current Sensor
  igbt_dyn : Subsystem
      settings: PortSchema="{\"entries\":[{\"content\":{\"sides\":[{\"content\":{\"connectorIds\":[\"LConn1\"]},\"type\":\"ConnectorPlacement.EquallySpacedRectSide\",\"uuid\":\"9362f9b7-ee93-45f5-82dd-187a901e7163\"},{\"content\":{\"side\":\"RIGHT\"},\"type\":\"ConnectorPlacement.EquallySpacedRectSide\",\"uuid\":\"6bcfd024-782a-41e2-b73d-7f1803740400\"},{\"content\":{\"connectorIds\":[\"LConn2\"],\"side\":\"TOP\"},\"type\":\"ConnectorPlacement.EquallySpacedRectSide\",\"uuid\":\"acf2fd2a-16ab-451c-9949-ad592b9336db\"},{\"content\":{\"connectorIds\":[\"RConn1\"],\"side\":\"BOTTOM\"},\"type\":\"ConnectorPlacement.EquallySpacedRectSide\",\"uuid\":\"befa74e7-1b93-47d7-b2f5-8e4e16cc48d3\"}]},\"type\":\"ConnectorPlacement.EquallySpacedConnector\",\"uuid\":\"1ef05993-5e93-4d63-8a9c-9607affd4d31\"}],\"packageUris\":[\"http://schema.mathworks.com/mf0/Connector/R2020b\"],\"version\":\"1.0\"}"
  iph1 : nesl_utility/PS-Simulink Converter  PhysicalDomain=network_engine_domain  SubClassName=ps_output  LeftPortType=input  RightPortType=output  PseudoPeriodic=off  Frequencies=[]  VectorFormat=1-D array  Unit=A  AffineConversion=off
  G : PMIOPort  Side=Left
  C : PMIOPort  Port=2  Side=Left
  E : PMIOPort  Port=3  Side=Right
  tag scope: igbt_current_Q2=scoped
  wires:
  iph1/1 -> [igbt_current_Q2]  "i_device_thermal_inv"
  connections:
  C/RConn1 -- Current Sensor/LConn1
  E/RConn1 -- igbt_dyn/RConn1
  Current Sensor/RConn2 -- igbt_dyn/LConn2
  iph1/LConn1 -- Current Sensor/RConn1
  G/RConn1 -- igbt_dyn/LConn1

== system dpt/dpt/leg/leg/leg_with_igbt_dyn/leg_with_igbt_dyn/igbt_dyn_1/IGBT_dyn/IGBT_dyn/IGBT_dyn/igbt_dyn ==
  IGBT (switching dynamics) : igbt_dyn_lib/IGBT (switching dynamics)  Vth=6.5 V  Kp=100 A/V^2  lam=0 1/V  Cge=180e-9 F  Cgc0=25e-9 F  Vjc=1 V  mc=0.7  Cce0=30e-9 F  Vjo=1 V  mo=0.5  Rg=1 Ohm  ftail=0.25  tauT=1.5e-6 s  dsm=0.5 V  ig_specify=off  ig_priority=None  ig=0 A  ig_nominal_specify=off  ig_nominal_value=1  ig_nominal_unit=A  ige_specify=off  ige_priority=None  ige=0 A  ige_nominal_specify=off  ige_nominal_value=1  ige_nominal_unit=A  igc_specify=off  igc_priority=None  igc=0 A  igc_nominal_specify=off  igc_nominal_value=1  igc_nominal_unit=A  ich_specify=off  ich_priority=None  ich=0 A  ich_nominal_specify=off  ich_nominal_value=1  ich_nominal_unit=A  icap_specify=off  icap_priority=None  icap=0 A  icap_nominal_specify=off  icap_nominal_value=1  icap_nominal_unit=A  itl_specify=off  itl_priority=None  itl=0 A  itl_nominal_specify=off  itl_nominal_value=1  itl_nominal_unit=A  vge_specify=off  vge_priority=None  vge=0 V  vge_nominal_specify=off  vge_nominal_value=1  vge_nominal_unit=V  vgc_specify=off  vgc_priority=None  vgc=0 V  vgc_nominal_specify=off  vgc_nominal_value=1  vgc_nominal_unit=V  vce_specify=off  vce_priority=None  vce=10 V  vce_nominal_specify=off  vce_nominal_value=1  vce_nominal_unit=V  qge_specify=off  qge_priority=None  qge=0 C  qge_nominal_specify=off  qge_nominal_value=1  qge_nominal_unit=C  qgc_specify=off  qgc_priority=None  qgc=0 C  qgc_nominal_specify=off  qgc_nominal_value=1  qgc_nominal_unit=C  qce_specify=off  qce_priority=None  qce=0 C  qce_nominal_specify=off  qce_nominal_value=1  qce_nominal_unit=C
  G : PMIOPort  Side=Left
  C : PMIOPort  Port=2  Side=Left
  E : PMIOPort  Port=3  Side=Right
  connections:
  IGBT (switching dynamics)/RConn2 -- E/RConn1
  IGBT (switching dynamics)/LConn1 -- G/RConn1
  IGBT (switching dynamics)/RConn1 -- C/RConn1

== system dpt/dpt/leg/leg/leg_with_igbt_dyn/leg_with_igbt_dyn/igbt_dyn_2/IGBT_dyn/IGBT_dyn/IGBT_dyn/igbt_dyn ==
  IGBT (switching dynamics) : igbt_dyn_lib/IGBT (switching dynamics)  Vth=6.5 V  Kp=100 A/V^2  lam=0 1/V  Cge=180e-9 F  Cgc0=25e-9 F  Vjc=1 V  mc=0.7  Cce0=30e-9 F  Vjo=1 V  mo=0.5  Rg=1 Ohm  ftail=0.25  tauT=1.5e-6 s  dsm=0.5 V  ig_specify=off  ig_priority=None  ig=0 A  ig_nominal_specify=off  ig_nominal_value=1  ig_nominal_unit=A  ige_specify=off  ige_priority=None  ige=0 A  ige_nominal_specify=off  ige_nominal_value=1  ige_nominal_unit=A  igc_specify=off  igc_priority=None  igc=0 A  igc_nominal_specify=off  igc_nominal_value=1  igc_nominal_unit=A  ich_specify=off  ich_priority=None  ich=0 A  ich_nominal_specify=off  ich_nominal_value=1  ich_nominal_unit=A  icap_specify=off  icap_priority=None  icap=0 A  icap_nominal_specify=off  icap_nominal_value=1  icap_nominal_unit=A  itl_specify=off  itl_priority=None  itl=0 A  itl_nominal_specify=off  itl_nominal_value=1  itl_nominal_unit=A  vge_specify=off  vge_priority=None  vge=0 V  vge_nominal_specify=off  vge_nominal_value=1  vge_nominal_unit=V  vgc_specify=off  vgc_priority=None  vgc=0 V  vgc_nominal_specify=off  vgc_nominal_value=1  vgc_nominal_unit=V  vce_specify=off  vce_priority=None  vce=10 V  vce_nominal_specify=off  vce_nominal_value=1  vce_nominal_unit=V  qge_specify=off  qge_priority=None  qge=0 C  qge_nominal_specify=off  qge_nominal_value=1  qge_nominal_unit=C  qgc_specify=off  qgc_priority=None  qgc=0 C  qgc_nominal_specify=off  qgc_nominal_value=1  qgc_nominal_unit=C  qce_specify=off  qce_priority=None  qce=0 C  qce_nominal_specify=off  qce_nominal_value=1  qce_nominal_unit=C
  G : PMIOPort  Side=Left
  C : PMIOPort  Port=2  Side=Left
  E : PMIOPort  Port=3  Side=Right
  connections:
  IGBT (switching dynamics)/RConn1 -- C/RConn1
  IGBT (switching dynamics)/LConn1 -- G/RConn1
  IGBT (switching dynamics)/RConn2 -- E/RConn1

== matlab function dpt/leg/leg/leg_pwm/modulator1/one phase PWM generator with global TRGO/MATLAB Function ==
  data: t input; y output; phase input; period input
function y = ramp_up_down(t,phase,period)
x = sin(2*pi/period*t - phase -pi/2);
y = asin(x)/pi + 1/2;
